simulink model "PitchSys"  (Simulink 8.4)
settings: Solver=ode1  StartTime=0.00  StopTime=10.00  FixedStep=0.01  RelTol=1e-3
settings Model: Creator=bjones  LastModifiedBy=bjones
settings DataIOCC: LimitDataPoints=off
settings OptimizationCC: BlockReduction=off  BooleanDataType=off
settings DebuggingCC: SaveWithParameterizedLinksMsg=none  SignalResolutionControl=TryResolveAllWithWarning  SolverPrmCheckMsg=none  MultiTaskDSMMsg=warning  MultiTaskCondExecSysMsg=none  StrictBusMsg=None
settings HardwareCC: TargetUnknown=on
settings RTWCC: IncludeERTFirstTime=on

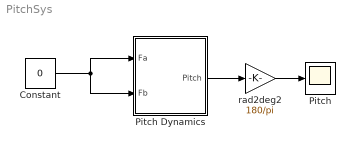
== system PitchSys ==
  Constant : Constant  Value=0
  Pitch : Scope
      settings: TimeRange=10  YMin=-30  YMax=30  SaveName=pitch
  Pitch Dynamics : Subsystem
  rad2deg2 : Gain  Gain=180/pi  SaturateOnIntegerOverflow=on  OutDataTypeStr=Inherit: Same as input  ParamDataTypeStr=Inherit: Same as input
  wires:
  Pitch Dynamics/1(Pitch) -> rad2deg2/1
  rad2deg2/1 -> Pitch/1
  Constant/1 -> Pitch Dynamics/1(Fa), Pitch Dynamics/2(Fb)

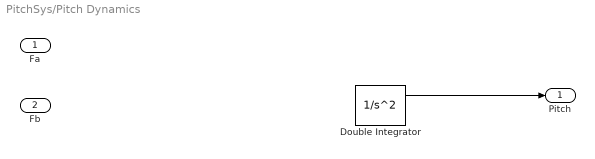
== system PitchSys/Pitch Dynamics ==
  Fa : Inport
  Fb : Inport  Port=2
  Double Integrator : SecondOrderIntegrator  ICX=p_lim_u  LimitX=on  UpperLimitX=p_lim_u  LowerLimitX=p_lim_l
  Pitch : Outport
  wires:
  Double Integrator/1 -> Pitch/1
